simulink model "s_aero2_2dof_pp"  (R2024b)
settings: Solver=ode4  StartTime=0.0  StopTime=30  FixedStep=0.002  RelTol=1e-3
values from neighbouring files (symbols this model uses):
  A = [0,       0,      1,      0 ... (first row only)    [aero2_2dof_control_pp.m]
  B = [0,            0 ... (first row only)    [aero2_2dof_control_pp.m]
  C = [1, 0, 0, 0 ... (first row only)    [aero2_2dof_control_pp.m]
  D = zeros(2, 2)    [aero2_2dof_control_pp.m]
  K = place(A, B, desired_poles)    [aero2_2dof_control_pp.m]
libraries: simulink_extras x4, quarc_library x2
settings Model: Creator=MLevis  LastModifiedBy=dinhck
settings DataIOCC: ReturnWorkspaceOutputs=off
settings DebuggingCC: UnconnectedInputMsg=warning  UnconnectedOutputMsg=warning  UnconnectedLineMsg=warning
settings ModelReferenceCC: EnableRefExpFcnMdlSchedulingChecks=on
settings RTWCC: GPUComputeCapability=3.5  DLArmComputeVersion=19.05

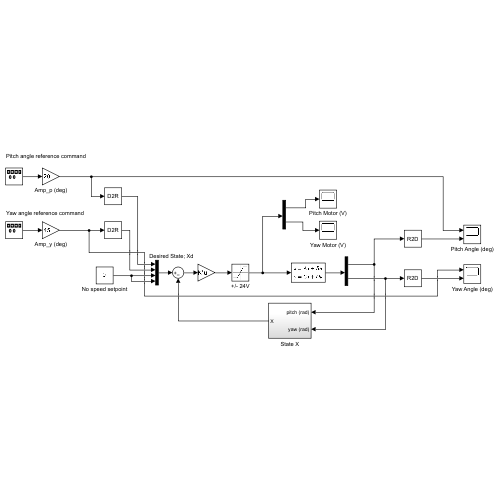
[thumbnail: Simulink's stored preview of the top-level diagram]
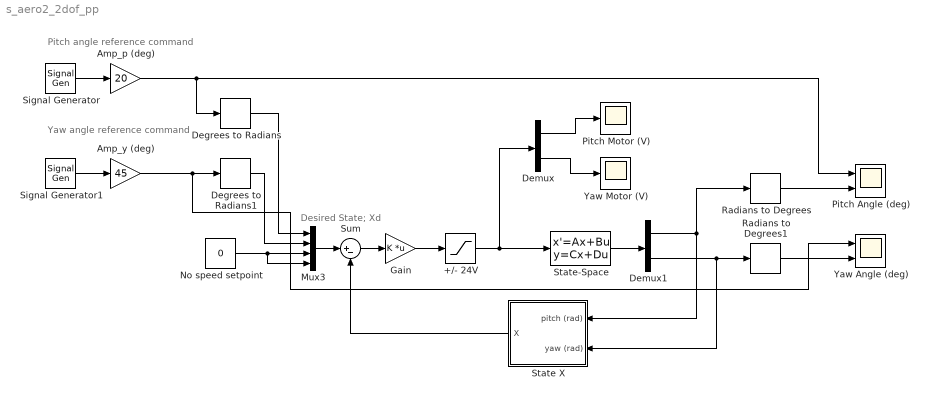
== system s_aero2_2dof_pp ==
  note: Pitch angle reference command
  note: Desired State; Xd
  note: Yaw angle reference command
  +/- 24V : Saturate  UpperLimit=24  LowerLimit=-24
  Amp_p (deg) : Gain  Gain=20
  Amp_y (deg) : Gain  Gain=45
  Degrees to Radians : simulink_extras/Transformations/Degrees to Radians
  Degrees to Radians1 : simulink_extras/Transformations/Degrees to Radians
  Demux : Demux  Outputs=2
  Demux1 : Demux  Outputs=2
  Gain : Gain  Gain=K  Multiplication=Matrix(K*u)
  Mux3 : Mux
  No speed setpoint : Constant  Value=0
  Pitch Angle (deg) : Scope  NumInputPorts=2
  Pitch Motor (V) : Scope
  Radians to Degrees : simulink_extras/Transformations/Radians to Degrees
  Radians to Degrees1 : simulink_extras/Transformations/Radians to Degrees
  Signal Generator : SignalGenerator  WaveForm=square  Frequency=0.05
  Signal Generator1 : SignalGenerator  WaveForm=square  Frequency=0.04
  State X : Subsystem
  State-Space : StateSpace  A=A  B=B  C=C  D=D  InitialCondition=0
  Sum : Sum  Inputs=|+-
  Yaw Angle (deg) : Scope  NumInputPorts=2
  Yaw Motor (V) : Scope
  wires:
  No speed setpoint/1 -> Mux3/4, Mux3/3
  Sum/1 -> Gain/1
  Demux1/2 -> Radians to Degrees1/1, State X/2(yaw (rad))
  Demux/2 -> Yaw Motor (V)/1
  +/- 24V/1 -> State-Space/1, Demux/1
  Signal Generator1/1 -> Amp_y (deg)/1
  Mux3/1 -> Sum/1
  State-Space/1 -> Demux1/1
  Demux1/1 -> Radians to Degrees/1, State X/1(pitch (rad))
  State X/1(X) -> Sum/2
  Demux/1 -> Pitch Motor (V)/1
  Gain/1 -> +/- 24V/1
  Amp_p (deg)/1 -> Pitch Angle (deg)/1, Degrees to Radians/1
  Signal Generator/1 -> Amp_p (deg)/1
  Amp_y (deg)/1 -> Yaw Angle (deg)/1, Degrees to Radians1/1
  Degrees to Radians/1 -> Mux3/1
  Degrees to Radians1/1 -> Mux3/2
  Radians to Degrees/1 -> Pitch Angle (deg)/2
  Radians to Degrees1/1 -> Yaw Angle (deg)/2

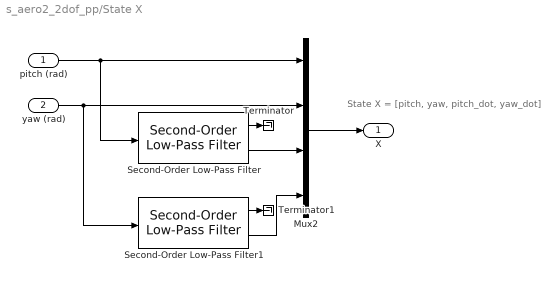
== system s_aero2_2dof_pp/State X ==
  note: State X = [pitch, yaw, pitch_dot, yaw_dot]
  pitch (rad) : Inport
  yaw (rad) : Inport  Port=2
  Mux2 : Mux
  Second-Order Low-Pass Filter : quarc_library/Continuous/Second-Order Low-Pass Filter  params_source=Internal (dialog parameters)  input_width=50  input_zeta=0.8  input_init=0
  Second-Order Low-Pass Filter1 : quarc_library/Continuous/Second-Order Low-Pass Filter  params_source=Internal (dialog parameters)  input_width=50  input_zeta=0.8  input_init=0
  Terminator : Terminator
  Terminator1 : Terminator
  X : Outport
  wires:
  Mux2/1 -> X/1
  yaw (rad)/1 -> Second-Order Low-Pass Filter1/1, Mux2/2
  pitch (rad)/1 -> Second-Order Low-Pass Filter/1, Mux2/1
  Second-Order Low-Pass Filter/2 -> Mux2/3
  Second-Order Low-Pass Filter1/2 -> Mux2/4
  Second-Order Low-Pass Filter/1 -> Terminator/1
  Second-Order Low-Pass Filter1/1 -> Terminator1/1
